simulink model "actualsystem"  (R2025a)
settings: Solver=VariableStepAuto  StartTime=0.0  StopTime=0.2  RelTol=1e-3
undefined symbols (not defined in the file): D11, Delta
libraries: spsRMSLib x9, spsCurrentMeasurementLib x4, spsACCurrentSourceLib x3, spsParallelRLCLoadLib x3, spsGroundLib x1, spsParallelRLCBranchLib x1, spsPower3phInstantaneousLib x1, spsThreePhasePISectionLineLib x1, spsThreePhaseSeriesRLCBranchLib x1, spsThreePhaseTransformerTwoWindingsLib x1, spsThreePhaseVIMeasurementLib x1, spsThreePhaseBreakerLib x1
settings Model: Creator=Krishna  LastModifiedBy=Ayush

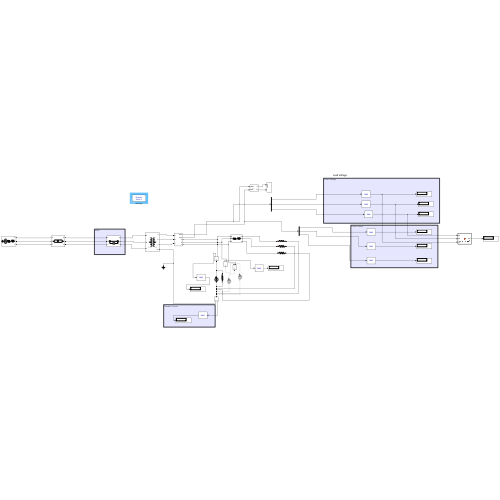
[thumbnail: Simulink's stored preview of the top-level diagram]
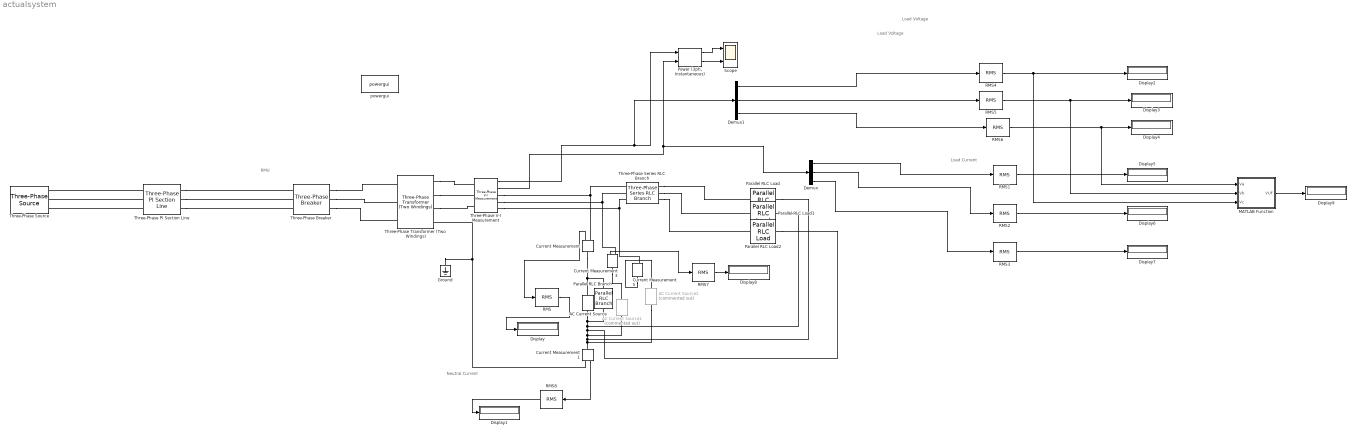
== system actualsystem ==
  note: RMU
  note: Load Current
  note: Load Voltage
  note: Load Voltage
  note: Neutral Current
  AC Current Source : spsACCurrentSourceLib/AC Current Source  Amplitude=20.86  Phase=-30  Frequency=50  SampleTime=0  Measurements=None
      settings: LibrarySourceBlock=sps_lib/Sources/AC Current Source
  AC Current Source1 : spsACCurrentSourceLib/AC Current Source  Commented=on  Amplitude=20.86  Phase=-150  Frequency=50  SampleTime=0  Measurements=None
      settings: LibrarySourceBlock=sps_lib/Sources/AC Current Source
  AC Current Source2 : spsACCurrentSourceLib/AC Current Source  Commented=on  Amplitude=20.86  Phase=90  Frequency=50  SampleTime=0  Measurements=None
      settings: LibrarySourceBlock=sps_lib/Sources/AC Current Source
  Current Measurement{,1,3,5} (4 alike) : spsCurrentMeasurementLib/Current Measurement  PhasorSimulation=off  OutputType=Complex  PSBequivalent=0
  Demux : Demux  Outputs=3
  Demux1 : Demux  Outputs=3
  Display{,1..9} (10 alike) : Display
  Ground : spsGroundLib/Ground  LConnTagsString=a
  MATLAB Function : MATLAB Function  TreatAsAtomicUnit=on
  Parallel RLC Branch : spsParallelRLCBranchLib/Parallel RLC Branch  LConnTagsString=a  RConnTagsString=__new0  BranchType=R  Resistance=1000000  Inductance=1e-3  SetiL0=off  InitialCurrent=0  Capacitance=1e-6  Setx0=off  InitialVoltage=0  Measurements=None
  Parallel RLC Load : spsParallelRLCLoadLib/Parallel RLC Load  LConnTagsString=a  RConnTagsString=__new0  NominalVoltage=239.6  NominalFrequency=50  ActivePower=10e3  InductivePower=0  CapacitivePower=0  Setx0=off  InitialVoltage=0  SetiL0=off  InitialCurrent=0  Measurements=None  LoadType=constant Z
      settings: AttributesFormatString=\n  LibrarySourceBlock=sps_lib/Passives/Parallel RLC Load
  Parallel RLC Load1 : spsParallelRLCLoadLib/Parallel RLC Load  LConnTagsString=a  RConnTagsString=__new0  NominalVoltage=239.6  NominalFrequency=50  ActivePower=13e3  InductivePower=0  CapacitivePower=0  Setx0=off  InitialVoltage=0  SetiL0=off  InitialCurrent=0  Measurements=None  LoadType=constant Z
      settings: AttributesFormatString=\n  LibrarySourceBlock=sps_lib/Passives/Parallel RLC Load
  Parallel RLC Load2 : spsParallelRLCLoadLib/Parallel RLC Load  LConnTagsString=a  RConnTagsString=__new0  NominalVoltage=239.6  NominalFrequency=50  ActivePower=18e3  InductivePower=0  CapacitivePower=0  Setx0=off  InitialVoltage=0  SetiL0=off  InitialCurrent=0  Measurements=None  LoadType=constant Z
      settings: AttributesFormatString=\n  LibrarySourceBlock=sps_lib/Passives/Parallel RLC Load
  "Power (3ph, Instantaneous)" : spsPower3phInstantaneousLib/Power (3ph, Instantaneous)
  RMS{,1..8} (9 alike) : spsRMSLib/RMS  TrueRMS=on  Freq=50  RMSInit=0  Ts=0
  Scope : Scope  NumInputPorts=2
  Three-Phase PI Section Line : spsThreePhasePISectionLineLib/Three-Phase PI Section Line  LConnTagsString=a|b|c  RConnTagsString=A|B|C  Length=10  Frequency=50  Resistances=[ 0.01273 0.3864]  Inductances="[ 0.9337e-3  4.1264e-3]"  Capacitances=[12.74e-9 7.751e-9]
  Three-Phase Series RLC Branch : spsThreePhaseSeriesRLCBranchLib/Three-Phase Series RLC Branch  LConnTagsString=A|B|C  RConnTagsString=A|B|C  BranchType=RL  Resistance=0.096  Inductance=0.0001  Capacitance=1e-6  Measurements=None
  Three-Phase Transformer (Two Windings) : spsThreePhaseTransformerTwoWindingsLib/Three-Phase Transformer (Two Windings)  Winding1Connection=Delta (D11)  Winding2Connection=Yn  CoreType=Three single-phase transformers  SetSaturation=off  Hysteresis=off  DataFile='hysteresis'  SetInitialFlux=off  Measurements=None  UNITS=pu  NominalPower=[ 315e3 , 50 ]  Winding1=[ 11000, 0.005 , 0.04]  Winding2=[ 415 , 0.005 , 0.04 ]  Rm=500  Lm=500  L0=0.5  Saturation=[ 0,0 ; 0.0024,1.2 ; 1.0,1.52 ]  InitialFluxes=[ 0.8 , -0.8 , 0.7 ]  BreakLoop=off  DiscreteSolver=Trapezoidal iterative  DataType=off  TransfoNumber=1
  Three-Phase V-I Measurement : spsThreePhaseVIMeasurementLib/Three-Phase V-I Measurement  VoltageMeasurement=phase-to-ground  SetLabelV=off  LabelV=Vabc  Vpu=off  VpuLL=off  CurrentMeasurement=yes  SetLabelI=off  LabelI=Iabc  Ipu=off  Pbase=100e6  Vbase=500e3  OutputType=Complex  PhasorSimulation=off  PSBequivalent=0
  Three-Phase Breaker : spsThreePhaseBreakerLib/Three-Phase Breaker  InitialState=closed  SwitchA=on  SwitchB=on  SwitchC=on  SwitchTimes="[1/60  5/60]"  External=off  BreakerResistance=0.01  SnubberResistance=1e6  SnubberCapacitance=inf  Measurements=None
  Three-Phase Source : spsThreePhaseSourceLib/Three-Phase Source  InternalConnection=Yg  VoltagePhases=off  Voltage=11000  PhaseAngle=0  Voltage_phases=[25e3 25e3 25e3]/sqrt(3)  PhaseAngles_phases=[0 -120 +120]  Frequency=50  NonIdealSource=on  SpecifyImpedance=on  Resistance=0.01  Inductance=0  ShortCircuitLevel=100e6  BaseVoltage=11e3  XRratio=7  BusType=swing  Pref=10e3  Qref=0  Prefabc=[10e3, 10e3, 10e3]  Qrefabc=[0, 0, 0]  Qmin=-inf  Qmax=inf
  powergui : sps_lib/powergui  Priority=1  SimulationMode=Discrete  SampleTime=50e-6  frequency=60  Iterations=50  frequencyindice=50  Pbase=100e6  ErrMax=1e-4  UnitsV=kV  UnitsW=MW  buscounter=0  FunctionMessages=off  echomessages=off  EnableUseOfTLC=off  CurrentSourceSwitches=off  DisableSnubberDevices=off  DisableRonSwitches=off  DisableVfSwitches=off  DisplayEquations=off  AutomaticDiscreteSolvers=off  SolverType=Tustin/Backward Euler (TBE)  Interpol=off  ExternalGateDelay=off  methode=off  Ts=100  x0status=blocks  SPID=on  SwTol=0  HookPort=off  NonlinearTolerance=1e-4  nMaxIteration=100  ContinueOnMaxIteration=off  RestoreLinks=warning  ResistiveCurrentMeasurement=off  Frange=[0:2:500]  Ylog=off  Xlog=on  ShowGrid=off  save=off  variable=ZData  structure=0  ZoomFFT=off  StartTime=0.0  cycles=1  DisplayStyle=1  fundamental=60  FreqAxis=off  MaxFrequency=1000  frequencyindicesteady=1  RmsSteady=1  display=off
  wires:
  Current Measurement/1 -> RMS/1
  RMS/1 -> Display/1
  Demux/1 -> RMS1/1
  Demux/2 -> RMS2/1
  Demux/3 -> RMS3/1
  Demux1/1 -> RMS4/1
  Demux1/2 -> RMS5/1
  Demux1/3 -> RMS6/1
  RMS4/1 -> MATLAB Function/3(Vc), Display2/1
  RMS5/1 -> MATLAB Function/2(Vb), Display3/1
  RMS6/1 -> MATLAB Function/1(Va), Display4/1
  "Power (3ph, Instantaneous)"/2 -> Scope/2
  "Power (3ph, Instantaneous)"/1 -> Scope/1
  RMS1/1 -> Display5/1
  RMS2/1 -> Display6/1
  RMS3/1 -> Display7/1
  Current Measurement3/1 -> RMS7/1
  RMS7/1 -> Display8/1
  Current Measurement1/1 -> RMS8/1
  RMS8/1 -> Display1/1
  MATLAB Function/1(VUF) -> Display9/1
  Three-Phase V-I Measurement/1 -> Demux1/1, "Power (3ph, Instantaneous)"/1
  Three-Phase V-I Measurement/2 -> Demux/1, "Power (3ph, Instantaneous)"/2
  connections:
  Three-Phase Breaker/RConn1 -- Three-Phase Transformer (Two Windings)/LConn1
  Three-Phase Breaker/RConn2 -- Three-Phase Transformer (Two Windings)/LConn2
  Three-Phase Breaker/RConn3 -- Three-Phase Transformer (Two Windings)/LConn3
  Current Measurement/RConn1 -- Three-Phase Series RLC Branch/LConn1 -- Three-Phase V-I Measurement/RConn1
  Current Measurement3/RConn1 -- Three-Phase V-I Measurement/RConn2 -- Three-Phase Series RLC Branch/LConn2
  Current Measurement5/RConn1 -- Three-Phase V-I Measurement/RConn3 -- Three-Phase Series RLC Branch/LConn3
  Three-Phase PI Section Line/LConn1 -- Three-Phase Source/RConn1
  Three-Phase PI Section Line/LConn2 -- Three-Phase Source/RConn2
  Three-Phase PI Section Line/LConn3 -- Three-Phase Source/RConn3
  Three-Phase PI Section Line/RConn1 -- Three-Phase Breaker/LConn1
  Three-Phase PI Section Line/RConn2 -- Three-Phase Breaker/LConn2
  Three-Phase PI Section Line/RConn3 -- Three-Phase Breaker/LConn3
  Current Measurement/LConn1 -- Parallel RLC Branch/LConn1 -- AC Current Source/RConn1
  AC Current Source/LConn1 -- Parallel RLC Branch/RConn1 -- Parallel RLC Load1/RConn1 -- Parallel RLC Load2/RConn1 -- AC Current Source1/LConn1 -- Parallel RLC Load/RConn1 -- AC Current Source2/LConn1 -- Current Measurement1/LConn1
  Current Measurement1/RConn1 -- Ground/LConn1 -- Three-Phase Transformer (Two Windings)/RConn4
  Current Measurement3/LConn1 -- AC Current Source1/RConn1
  Current Measurement5/LConn1 -- AC Current Source2/RConn1
  Three-Phase Series RLC Branch/RConn1 -- Parallel RLC Load/LConn1
  Three-Phase Series RLC Branch/RConn2 -- Parallel RLC Load1/LConn1
  Three-Phase Series RLC Branch/RConn3 -- Parallel RLC Load2/LConn1
  Three-Phase Transformer (Two Windings)/RConn1 -- Three-Phase V-I Measurement/LConn1
  Three-Phase Transformer (Two Windings)/RConn2 -- Three-Phase V-I Measurement/LConn2
  Three-Phase Transformer (Two Windings)/RConn3 -- Three-Phase V-I Measurement/LConn3

== matlab function actualsystem/MATLAB Function ==
  data: Va input; VUF output; Vb input; Vc input
function VUF = compute_vuf(Va, Vb, Vc)
Vavg = (abs(Va) + abs(Vb) + abs(Vc)) / 3;
VUF = max([abs(abs(Va)-Vavg), ...
           abs(abs(Vb)-Vavg), ...
           abs(abs(Vc)-Vavg)]) / Vavg * 100;
end
